simulink model "fulladder"  (R2022b)
settings: Solver=VariableStepAuto  StartTime=0.0  StopTime=10.0  RelTol=1e-3
settings Model: Creator=shaibalsaha  LastModifiedBy=shaibalsaha

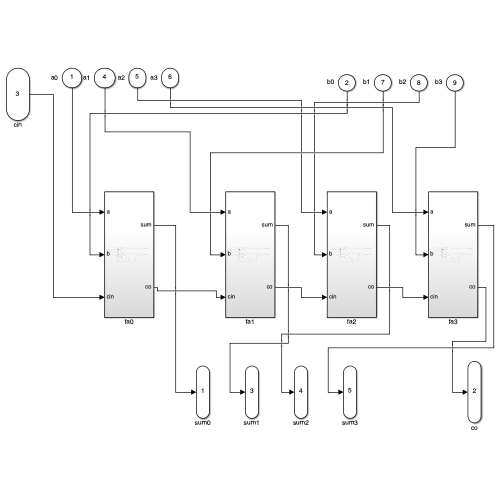
[thumbnail: Simulink's stored preview of the top-level diagram]
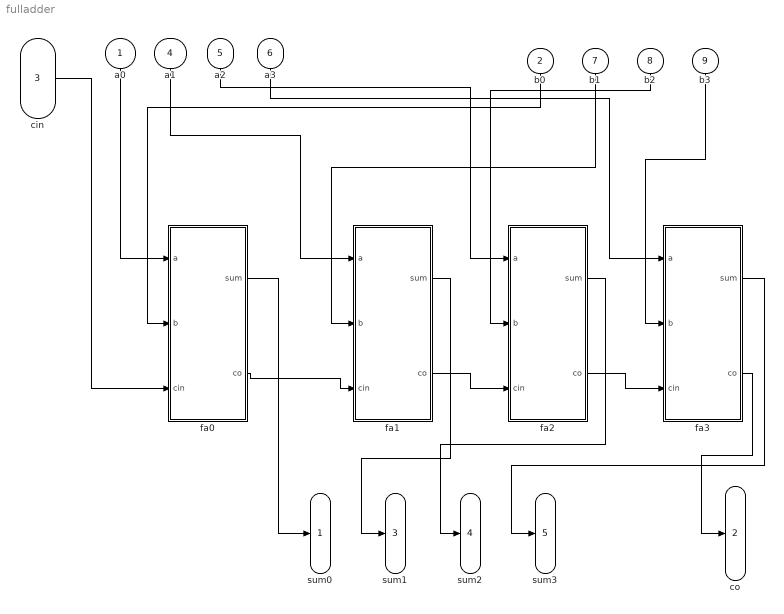
== system fulladder ==
  a0 : Inport
  b0 : Inport  Port=2
  cin : Inport  Port=3
  a1 : Inport  Port=4
  a2 : Inport  Port=5
  a3 : Inport  Port=6
  b1 : Inport  Port=7
  b2 : Inport  Port=8
  b3 : Inport  Port=9
  fa0 : Subsystem
  fa1 : Subsystem
  fa2 : Subsystem
  fa3 : Subsystem
  sum0 : Outport  VectorParamsAs1DForOutWhenUnconnected=off
  co : Outport  Port=2  VectorParamsAs1DForOutWhenUnconnected=off
  sum1 : Outport  Port=3  VectorParamsAs1DForOutWhenUnconnected=off
  sum2 : Outport  Port=4  VectorParamsAs1DForOutWhenUnconnected=off
  sum3 : Outport  Port=5  VectorParamsAs1DForOutWhenUnconnected=off
  wires:
  a0/1 -> fa0/1(a)
  b0/1 -> fa0/2(b)
  cin/1 -> fa0/3(cin)
  fa0/1(sum) -> sum0/1
  fa0/2(co) -> fa1/3(cin)
  a1/1 -> fa1/1(a)
  b1/1 -> fa1/2(b)
  fa1/2(co) -> fa2/3(cin)
  fa2/2(co) -> fa3/3(cin)
  a2/1 -> fa2/1(a)
  b2/1 -> fa2/2(b)
  b3/1 -> fa3/2(b)
  a3/1 -> fa3/1(a)
  fa1/1(sum) -> sum1/1
  fa2/1(sum) -> sum2/1
  fa3/1(sum) -> sum3/1
  fa3/2(co) -> co/1

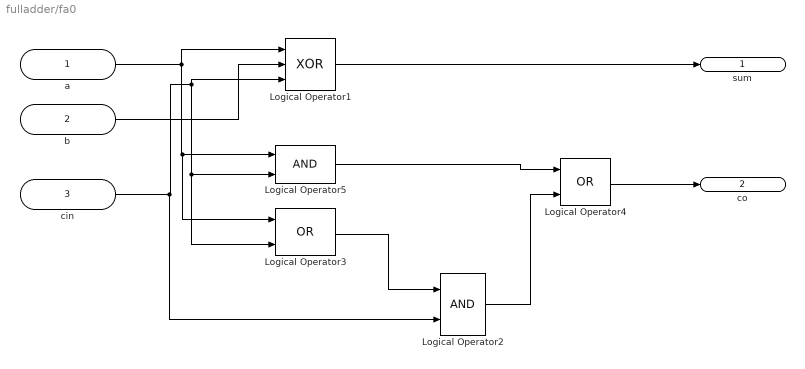
== system fulladder/fa0 ==
  a : Inport
  b : Inport  Port=2
  cin : Inport  Port=3
  Logical Operator1 : Logic  Operator=XOR  Inputs=3  AllPortsSameDT=off  OutDataTypeStr=boolean
  Logical Operator2 : Logic  AllPortsSameDT=off  OutDataTypeStr=boolean
  Logical Operator3 : Logic  Operator=OR  AllPortsSameDT=off  OutDataTypeStr=boolean
  Logical Operator4 : Logic  Operator=OR  AllPortsSameDT=off  OutDataTypeStr=boolean
  Logical Operator5 : Logic  AllPortsSameDT=off  OutDataTypeStr=boolean
  sum : Outport  VectorParamsAs1DForOutWhenUnconnected=off
  co : Outport  Port=2  VectorParamsAs1DForOutWhenUnconnected=off
  wires:
  b/1 -> Logical Operator1/2
  Logical Operator4/1 -> co/1
  Logical Operator3/1 -> Logical Operator2/1
  Logical Operator5/1 -> Logical Operator4/1
  Logical Operator2/1 -> Logical Operator4/2
  cin/1 -> Logical Operator2/2, Logical Operator1/3, Logical Operator5/2, Logical Operator3/2
  Logical Operator1/1 -> sum/1
  a/1 -> Logical Operator1/1, Logical Operator5/1, Logical Operator3/1

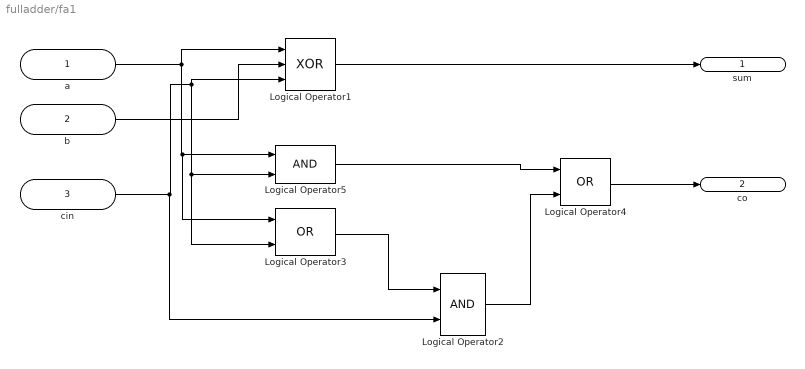
== system fulladder/fa1 ==
  a : Inport
  b : Inport  Port=2
  cin : Inport  Port=3
  Logical Operator1 : Logic  Operator=XOR  Inputs=3  AllPortsSameDT=off  OutDataTypeStr=boolean
  Logical Operator2 : Logic  AllPortsSameDT=off  OutDataTypeStr=boolean
  Logical Operator3 : Logic  Operator=OR  AllPortsSameDT=off  OutDataTypeStr=boolean
  Logical Operator4 : Logic  Operator=OR  AllPortsSameDT=off  OutDataTypeStr=boolean
  Logical Operator5 : Logic  AllPortsSameDT=off  OutDataTypeStr=boolean
  sum : Outport  VectorParamsAs1DForOutWhenUnconnected=off
  co : Outport  Port=2  VectorParamsAs1DForOutWhenUnconnected=off
  wires:
  b/1 -> Logical Operator1/2
  Logical Operator4/1 -> co/1
  Logical Operator3/1 -> Logical Operator2/1
  Logical Operator5/1 -> Logical Operator4/1
  Logical Operator2/1 -> Logical Operator4/2
  cin/1 -> Logical Operator2/2, Logical Operator1/3, Logical Operator5/2, Logical Operator3/2
  Logical Operator1/1 -> sum/1
  a/1 -> Logical Operator1/1, Logical Operator5/1, Logical Operator3/1

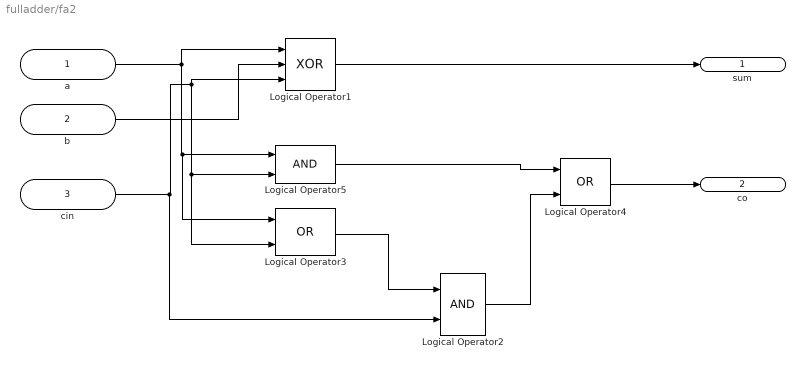
== system fulladder/fa2 ==
  a : Inport
  b : Inport  Port=2
  cin : Inport  Port=3
  Logical Operator1 : Logic  Operator=XOR  Inputs=3  AllPortsSameDT=off  OutDataTypeStr=boolean
  Logical Operator2 : Logic  AllPortsSameDT=off  OutDataTypeStr=boolean
  Logical Operator3 : Logic  Operator=OR  AllPortsSameDT=off  OutDataTypeStr=boolean
  Logical Operator4 : Logic  Operator=OR  AllPortsSameDT=off  OutDataTypeStr=boolean
  Logical Operator5 : Logic  AllPortsSameDT=off  OutDataTypeStr=boolean
  sum : Outport  VectorParamsAs1DForOutWhenUnconnected=off
  co : Outport  Port=2  VectorParamsAs1DForOutWhenUnconnected=off
  wires:
  b/1 -> Logical Operator1/2
  Logical Operator4/1 -> co/1
  Logical Operator3/1 -> Logical Operator2/1
  Logical Operator5/1 -> Logical Operator4/1
  Logical Operator2/1 -> Logical Operator4/2
  cin/1 -> Logical Operator2/2, Logical Operator1/3, Logical Operator5/2, Logical Operator3/2
  Logical Operator1/1 -> sum/1
  a/1 -> Logical Operator1/1, Logical Operator5/1, Logical Operator3/1

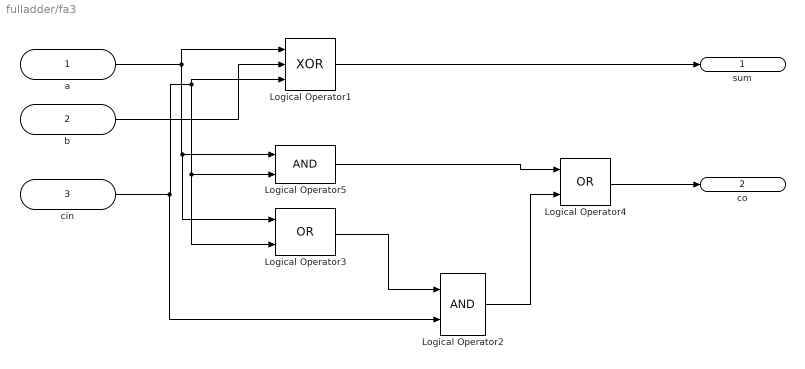
== system fulladder/fa3 ==
  a : Inport
  b : Inport  Port=2
  cin : Inport  Port=3
  Logical Operator1 : Logic  Operator=XOR  Inputs=3  AllPortsSameDT=off  OutDataTypeStr=boolean
  Logical Operator2 : Logic  AllPortsSameDT=off  OutDataTypeStr=boolean
  Logical Operator3 : Logic  Operator=OR  AllPortsSameDT=off  OutDataTypeStr=boolean
  Logical Operator4 : Logic  Operator=OR  AllPortsSameDT=off  OutDataTypeStr=boolean
  Logical Operator5 : Logic  AllPortsSameDT=off  OutDataTypeStr=boolean
  sum : Outport  VectorParamsAs1DForOutWhenUnconnected=off
  co : Outport  Port=2  VectorParamsAs1DForOutWhenUnconnected=off
  wires:
  b/1 -> Logical Operator1/2
  Logical Operator4/1 -> co/1
  Logical Operator3/1 -> Logical Operator2/1
  Logical Operator5/1 -> Logical Operator4/1
  Logical Operator2/1 -> Logical Operator4/2
  cin/1 -> Logical Operator2/2, Logical Operator1/3, Logical Operator5/2, Logical Operator3/2
  Logical Operator1/1 -> sum/1
  a/1 -> Logical Operator1/1, Logical Operator5/1, Logical Operator3/1
